simulink model "Energy_Management_Model1"  (R2025a)
settings: Solver=ode4  StartTime=0.0  StopTime=86400  FixedStep=3600  RelTol=1e-3
values from neighbouring files (symbols this model uses):
  A = 150    [setup_parameters.m]
  C_bat = 10    [setup_parameters.m]
  eta = 0.18    [setup_parameters.m]
  P_bat_max = 2    [setup_parameters.m]
  SOC_init = [0.3, 0.6, 0.9]    [setup_parameters.m]
  SOC_max = 0.98    [setup_parameters.m]
  SOC_min = 0.2    [setup_parameters.m]
  Ts = 3600    [setup_parameters.m]
libraries: simulink x3
settings Model: Creator=ENG HOSAM  LastModifiedBy=mtabrez
settings SolverCC: AlgebraicLoopSolver=TrustRegion
settings DebuggingCC: UnconnectedInputMsg=warning  UnconnectedOutputMsg=warning  UnconnectedLineMsg=warning
settings ModelReferenceCC: EnableRefExpFcnMdlSchedulingChecks=on
settings RTWCC: GPUComputeCapability=3.5

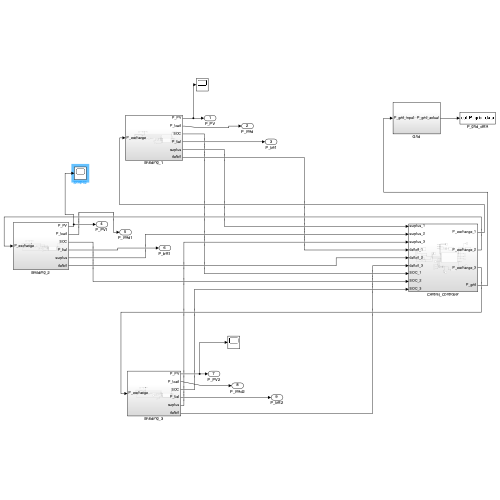
[thumbnail: Simulink's stored preview of the top-level diagram]
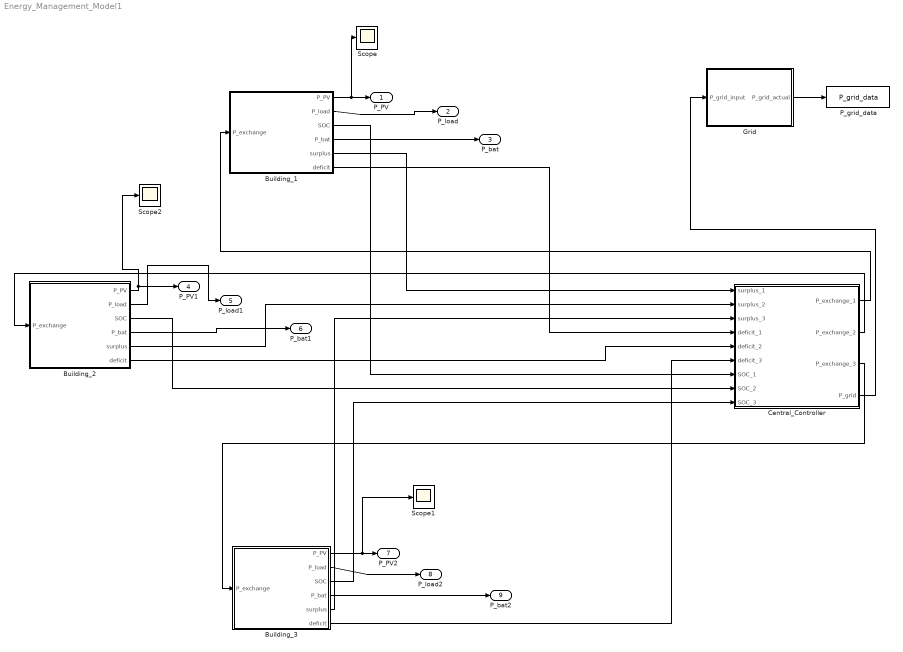
== system Energy_Management_Model1 ==
  Building_1 : Subsystem
  Building_2 : Subsystem
  Building_3 : Subsystem
  Central_Controller : Subsystem
  Grid : Subsystem
  P_grid_data : ToWorkspace  VariableName=P_grid_data  SampleTime=-1
  Scope : Scope
      settings: ActiveDisplayYMinimum=-3.3749999999999991  ActiveDisplayYMaximum=30.375  DataLoggingVariableName=ScopeData5
  Scope1 : Scope
      settings: DataLoggingVariableName=ScopeData6
  Scope2 : Scope
      settings: ActiveDisplayYMinimum=-3.3749999999999991  ActiveDisplayYMaximum=30.375  DataLoggingVariableName=ScopeData7
  P_PV : Outport
  P_load : Outport  Port=2
  P_bat : Outport  Port=3
  P_PV1 : Outport  Port=4
  P_load1 : Outport  Port=5
  P_bat1 : Outport  Port=6
  P_PV2 : Outport  Port=7
  P_load2 : Outport  Port=8
  P_bat2 : Outport  Port=9
  wires:
  Building_1/1(P_PV) -> Scope/1, P_PV/1
  Building_1/2(P_load) -> P_load/1
  Building_1/4(P_bat) -> P_bat/1
  Building_2/4(P_bat) -> P_bat1/1
  Building_2/1(P_PV) -> P_PV1/1, Scope2/1
  Building_2/2(P_load) -> P_load1/1
  Building_3/4(P_bat) -> P_bat2/1
  Building_3/1(P_PV) -> Scope1/1, P_PV2/1
  Building_3/2(P_load) -> P_load2/1
  Building_1/5(surplus) -> Central_Controller/1(surplus_1)
  Building_2/5(surplus) -> Central_Controller/2(surplus_2)
  Building_3/5(surplus) -> Central_Controller/3(surplus_3)
  Building_1/6(deficit) -> Central_Controller/4(deficit_1)
  Building_2/6(deficit) -> Central_Controller/5(deficit_2)
  Building_3/6(deficit) -> Central_Controller/6(deficit_3)
  Building_1/3(SOC) -> Central_Controller/7(SOC_1)
  Building_2/3(SOC) -> Central_Controller/8(SOC_2)
  Building_3/3(SOC) -> Central_Controller/9(SOC_3)
  Central_Controller/1(P_exchange_1) -> Building_1/1(P_exchange)
  Central_Controller/2(P_exchange_2) -> Building_2/1(P_exchange)
  Central_Controller/3(P_exchange_3) -> Building_3/1(P_exchange)
  Central_Controller/4(P_grid) -> Grid/1(P_grid_input)
  Grid/1(P_grid_actual) -> P_grid_data/1

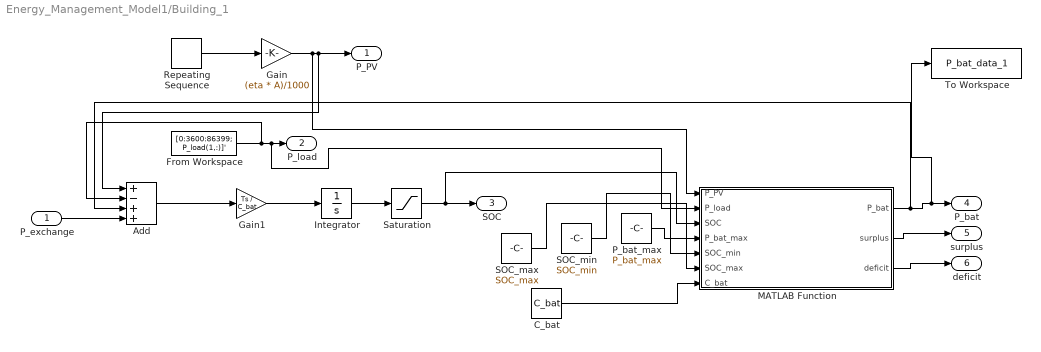
== system Energy_Management_Model1/Building_1 ==
  P_exchange : Inport
  Add : Sum  Inputs=+-++
  C_bat : Constant  Value=C_bat
  From Workspace : FromWorkspace  VariableName=[0:3600:86399; P_load(1,:)]'  OutDataTypeStr=double
  Gain : Gain  Gain=(eta * A)/1000
  Gain1 : Gain  Gain=Ts / C_bat
  Integrator : Integrator  InitialCondition=SOC_init(1)
  MATLAB Function : MATLAB Function  TreatAsAtomicUnit=on
  P_bat_max : Constant  Value=P_bat_max
  Repeating Sequence : simulink/Sources/Repeating Sequence  rep_seq_t=0:3600:82800  rep_seq_y=G
  SOC_max : Constant  Value=SOC_max
  SOC_min : Constant  Value=SOC_min
  Saturation : Saturate  UpperLimit=SOC_max  LowerLimit=SOC_min
  To Workspace : ToWorkspace  VariableName=P_bat_data_1  SampleTime=-1
  P_PV : Outport
  P_load : Outport  Port=2
  SOC : Outport  Port=3
  P_bat : Outport  Port=4
  surplus : Outport  Port=5
  deficit : Outport  Port=6
  wires:
  Integrator/1 -> Saturation/1
  MATLAB Function/3(deficit) -> deficit/1
  Gain1/1 -> Integrator/1
  From Workspace/1 -> Add/2, P_load/1, MATLAB Function/2(P_load)
  Gain/1 -> Add/1, P_PV/1, MATLAB Function/1(P_PV)
  Repeating Sequence/1 -> Gain/1
  Saturation/1 -> SOC/1, MATLAB Function/3(SOC)
  P_bat_max/1 -> MATLAB Function/4(P_bat_max)
  MATLAB Function/1(P_bat) -> Add/3, To Workspace/1, P_bat/1
  MATLAB Function/2(surplus) -> surplus/1
  SOC_max/1 -> MATLAB Function/6(SOC_max)
  SOC_min/1 -> MATLAB Function/5(SOC_min)
  C_bat/1 -> MATLAB Function/7(C_bat)
  Add/1 -> Gain1/1
  P_exchange/1 -> Add/4

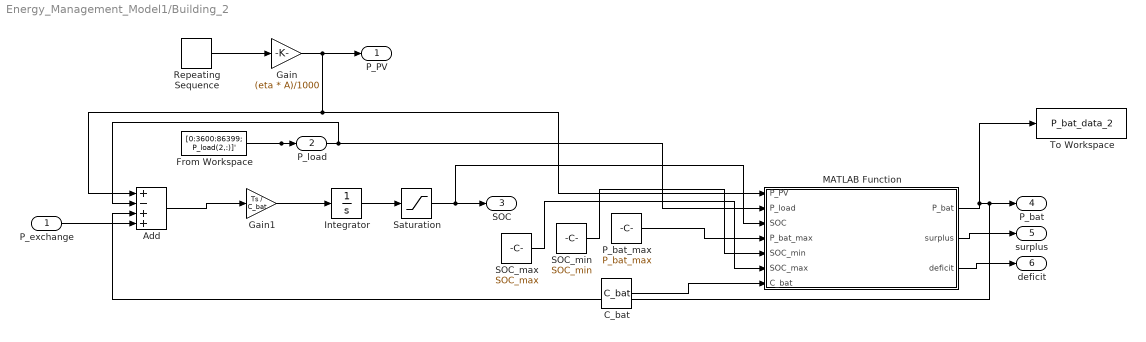
== system Energy_Management_Model1/Building_2 ==
  P_exchange : Inport
  Add : Sum  Inputs=+-++
  C_bat : Constant  Value=C_bat
  From Workspace : FromWorkspace  VariableName=[0:3600:86399; P_load(2,:)]'  OutDataTypeStr=double
  Gain : Gain  Gain=(eta * A)/1000
  Gain1 : Gain  Gain=Ts / C_bat
  Integrator : Integrator  InitialCondition=SOC_init(2)
  MATLAB Function : MATLAB Function  TreatAsAtomicUnit=on
  P_bat_max : Constant  Value=P_bat_max
  Repeating Sequence : simulink/Sources/Repeating Sequence  rep_seq_t=0:3600:82800  rep_seq_y=G
  SOC_max : Constant  Value=SOC_max
  SOC_min : Constant  Value=SOC_min
  Saturation : Saturate  UpperLimit=SOC_max  LowerLimit=SOC_min
  To Workspace : ToWorkspace  VariableName=P_bat_data_2  SampleTime=-1
  P_PV : Outport
  P_load : Outport  Port=2
  SOC : Outport  Port=3
  P_bat : Outport  Port=4
  surplus : Outport  Port=5
  deficit : Outport  Port=6
  wires:
  Integrator/1 -> Saturation/1
  MATLAB Function/3(deficit) -> deficit/1
  MATLAB Function/1(P_bat) -> To Workspace/1, Add/3, P_bat/1
  Gain1/1 -> Integrator/1
  From Workspace/1 -> P_load/1, Add/2, MATLAB Function/2(P_load)
  Gain/1 -> P_PV/1, Add/1, MATLAB Function/1(P_PV)
  Repeating Sequence/1 -> Gain/1
  Saturation/1 -> SOC/1, MATLAB Function/3(SOC)
  P_bat_max/1 -> MATLAB Function/4(P_bat_max)
  Add/1 -> Gain1/1
  MATLAB Function/2(surplus) -> surplus/1
  SOC_max/1 -> MATLAB Function/6(SOC_max)
  SOC_min/1 -> MATLAB Function/5(SOC_min)
  P_exchange/1 -> Add/4
  C_bat/1 -> MATLAB Function/7(C_bat)

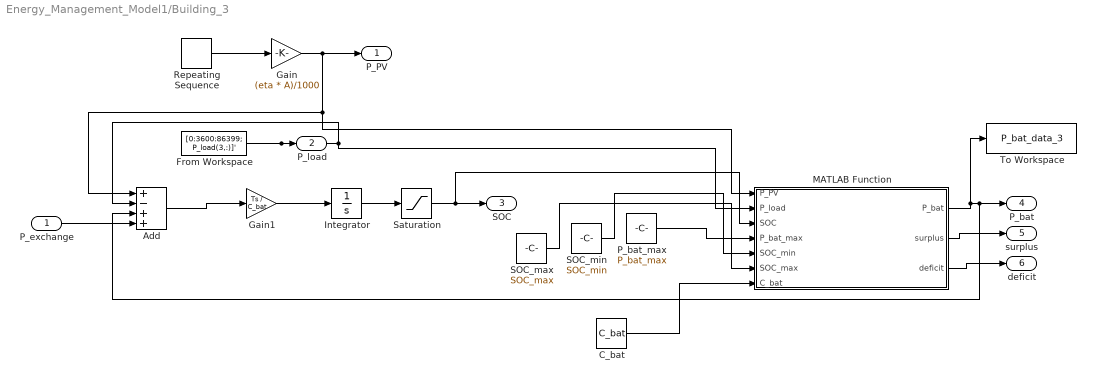
== system Energy_Management_Model1/Building_3 ==
  P_exchange : Inport
  Add : Sum  Inputs=+-++
  C_bat : Constant  Value=C_bat
  From Workspace : FromWorkspace  VariableName=[0:3600:86399; P_load(3,:)]'  OutDataTypeStr=double
  Gain : Gain  Gain=(eta * A)/1000
  Gain1 : Gain  Gain=Ts / C_bat
  Integrator : Integrator  InitialCondition=SOC_init(3)
  MATLAB Function : MATLAB Function  TreatAsAtomicUnit=on
  P_bat_max : Constant  Value=P_bat_max
  Repeating Sequence : simulink/Sources/Repeating Sequence  rep_seq_t=0:3600:82800  rep_seq_y=G
  SOC_max : Constant  Value=SOC_max
  SOC_min : Constant  Value=SOC_min
  Saturation : Saturate  UpperLimit=SOC_max  LowerLimit=SOC_min
  To Workspace : ToWorkspace  VariableName=P_bat_data_3  SampleTime=-1
  P_PV : Outport
  P_load : Outport  Port=2
  SOC : Outport  Port=3
  P_bat : Outport  Port=4
  surplus : Outport  Port=5
  deficit : Outport  Port=6
  wires:
  Integrator/1 -> Saturation/1
  MATLAB Function/3(deficit) -> deficit/1
  MATLAB Function/1(P_bat) -> To Workspace/1, Add/3, P_bat/1
  Gain1/1 -> Integrator/1
  From Workspace/1 -> P_load/1, Add/2, MATLAB Function/2(P_load)
  Gain/1 -> P_PV/1, Add/1, MATLAB Function/1(P_PV)
  Repeating Sequence/1 -> Gain/1
  Saturation/1 -> SOC/1, MATLAB Function/3(SOC)
  P_bat_max/1 -> MATLAB Function/4(P_bat_max)
  Add/1 -> Gain1/1
  MATLAB Function/2(surplus) -> surplus/1
  SOC_max/1 -> MATLAB Function/6(SOC_max)
  SOC_min/1 -> MATLAB Function/5(SOC_min)
  P_exchange/1 -> Add/4
  C_bat/1 -> MATLAB Function/7(C_bat)

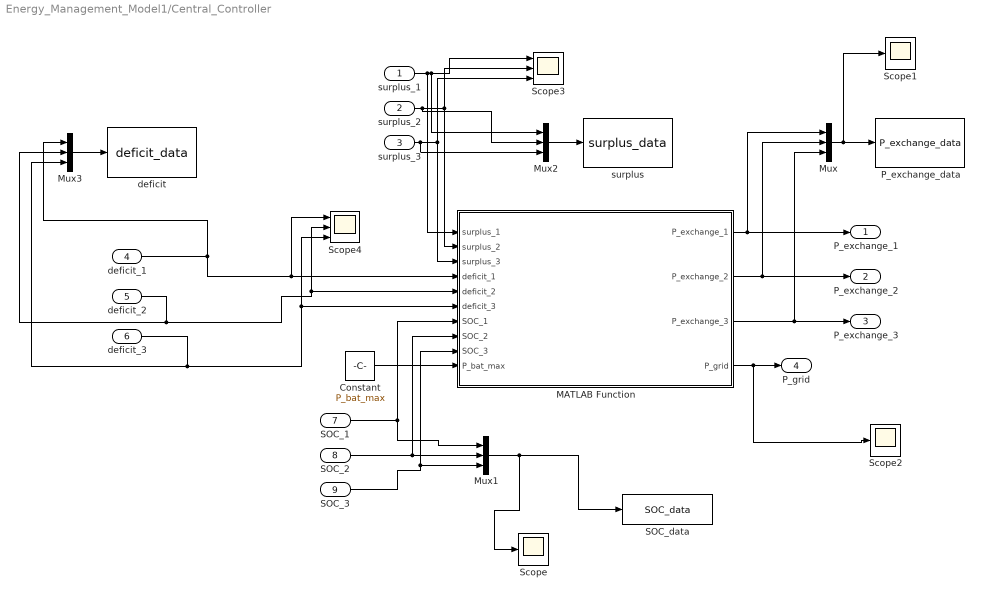
== system Energy_Management_Model1/Central_Controller ==
  surplus_1 : Inport
  surplus_2 : Inport  Port=2
  surplus_3 : Inport  Port=3
  deficit_1 : Inport  Port=4
  deficit_2 : Inport  Port=5
  deficit_3 : Inport  Port=6
  SOC_1 : Inport  Port=7
  SOC_2 : Inport  Port=8
  SOC_3 : Inport  Port=9
  Constant : Constant  Value=P_bat_max
  MATLAB Function : MATLAB Function  TreatAsAtomicUnit=on
  Mux{,1..3} (4 alike) : Mux  Inputs=3
  P_exchange_data : ToWorkspace  VariableName=P_exchange_data  SampleTime=-1
  SOC_data : ToWorkspace  VariableName=SOC_data  SampleTime=-1
  Scope : Scope
      settings: ActiveDisplayYMinimum=0.1025  ActiveDisplayYMaximum=1.0775
  Scope1 : Scope
      settings: ActiveDisplayYMinimum=-0.25  ActiveDisplayYMaximum=2.25
  Scope2 : Scope
      settings: ActiveDisplayYMinimum=-16.425  ActiveDisplayYMaximum=87.825  DataLoggingVariableName=ScopeData2
  Scope3 : Scope  NumInputPorts=3
      settings: ActiveDisplayYMinimum=-3.2375  ActiveDisplayYMaximum=29.1375  DataLoggingVariableName=ScopeData3
  Scope4 : Scope  NumInputPorts=3
      settings: ActiveDisplayYMinimum=-0.275  ActiveDisplayYMaximum=2.475  DataLoggingVariableName=ScopeData4
  deficit : ToWorkspace  VariableName=deficit_data  SampleTime=-1
  surplus : ToWorkspace  VariableName=surplus_data  SampleTime=-1
  P_exchange_1 : Outport
  P_exchange_2 : Outport  Port=2
  P_exchange_3 : Outport  Port=3
  P_grid : Outport  Port=4
  wires:
  SOC_2/1 -> MATLAB Function/8(SOC_2), Mux1/2
  SOC_1/1 -> MATLAB Function/7(SOC_1), Mux1/1
  MATLAB Function/1(P_exchange_1) -> Mux/1, P_exchange_1/1
  SOC_3/1 -> MATLAB Function/9(SOC_3), Mux1/3
  Mux1/1 -> Scope/1, SOC_data/1
  MATLAB Function/3(P_exchange_3) -> Mux/3, P_exchange_3/1
  MATLAB Function/2(P_exchange_2) -> Mux/2, P_exchange_2/1
  Mux/1 -> Scope1/1, P_exchange_data/1
  surplus_2/1 -> Mux2/2, Scope3/2, MATLAB Function/2(surplus_2)
  surplus_3/1 -> Mux2/3, Scope3/3, MATLAB Function/3(surplus_3)
  deficit_1/1 -> Mux3/1, Scope4/1, MATLAB Function/4(deficit_1)
  deficit_2/1 -> Scope4/2, MATLAB Function/5(deficit_2), Mux3/2
  deficit_3/1 -> MATLAB Function/6(deficit_3), Scope4/3, Mux3/3
  MATLAB Function/4(P_grid) -> Scope2/1, P_grid/1
  surplus_1/1 -> Mux2/1, Scope3/1, MATLAB Function/1(surplus_1)
  Mux2/1 -> surplus/1
  Mux3/1 -> deficit/1
  Constant/1 -> MATLAB Function/10(P_bat_max)

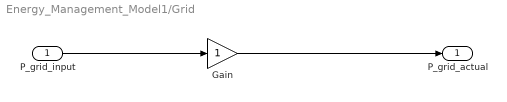
== system Energy_Management_Model1/Grid ==
  P_grid_input : Inport
  Gain : Gain
  P_grid_actual : Outport
  wires:
  P_grid_input/1 -> Gain/1
  Gain/1 -> P_grid_actual/1

== matlab function Energy_Management_Model1/Building_2/MATLAB Function ==
  data: P_PV input; P_bat output; P_load input; SOC input; P_bat_max input; SOC_min input; SOC_max input; surplus output; deficit output; C_bat input
function [P_bat, surplus, deficit] = local_controller(P_PV, P_load, SOC, P_bat_max, SOC_min, SOC_max, C_bat)
    net_power = P_PV - P_load;
    P_bat = 0;
    surplus = 0;
    deficit = 0;
    
    if net_power > 0
        if SOC < 0.8 && SOC < 0.98
            max_charge = min(P_bat_max, (SOC_max - SOC) * C_bat);
            P_bat = min(net_power, max_charge);
        end
        surplus = max(0, net_power - P_bat);
    elseif net_power < 0
        if SOC > 0.3 || (SOC > 0.7 && net_power < -0.1)
            max_discharge = min(P_bat_max, (SOC - SOC_min) * C_bat);
            P_bat = max(net_power, -max_discharge);
        end
        deficit = max(0, -net_power - P_bat);
    end
end

== matlab function Energy_Management_Model1/Building_1/MATLAB Function ==
  data: P_PV input; P_bat output; P_load input; SOC input; P_bat_max input; SOC_min input; SOC_max input; surplus output; deficit output; C_bat input
function [P_bat, surplus, deficit] = local_controller(P_PV, P_load, SOC, P_bat_max, SOC_min, SOC_max, C_bat)
    net_power = P_PV - P_load;
    P_bat = 0;
    surplus = 0;
    deficit = 0;
    
    if net_power > 0
        if SOC < 0.8 && SOC < 0.98
            max_charge = min(P_bat_max, (SOC_max - SOC) * C_bat);
            P_bat = min(net_power, max_charge);
        end
        surplus = max(0, net_power - P_bat);
    elseif net_power < 0
        if SOC > 0.3 || (SOC > 0.7 && net_power < -0.1)
            max_discharge = min(P_bat_max, (SOC - SOC_min) * C_bat);
            P_bat = max(net_power, -max_discharge);
        end
        deficit = max(0, -net_power - P_bat);
    end
end

== matlab function Energy_Management_Model1/Building_3/MATLAB Function ==
  data: P_PV input; P_bat output; P_load input; SOC input; P_bat_max input; SOC_min input; SOC_max input; surplus output; deficit output; C_bat input
function [P_bat, surplus, deficit] = local_controller(P_PV, P_load, SOC, P_bat_max, SOC_min, SOC_max, C_bat)
    net_power = P_PV - P_load;
    P_bat = 0;
    surplus = 0;
    deficit = 0;
    
    if net_power > 0
        if SOC < 0.8 && SOC < 0.98
            max_charge = min(P_bat_max, (SOC_max - SOC) * C_bat);
            P_bat = min(net_power, max_charge);
        end
        surplus = max(0, net_power - P_bat);
    elseif net_power < 0
        if SOC > 0.3 || (SOC > 0.7 && net_power < -0.1)
            max_discharge = min(P_bat_max, (SOC - SOC_min) * C_bat);
            P_bat = max(net_power, -max_discharge);
        end
        deficit = max(0, -net_power - P_bat);
    end
end

== matlab function Energy_Management_Model1/Central_Controller/MATLAB Function ==
  data: surplus_1 input; P_exchange_1 output; P_exchange_2 output; P_exchange_3 output; surplus_2 input; surplus_3 input; deficit_1 input; deficit_2 input; deficit_3 input; SOC_1 input; SOC_2 input; SOC_3 input; P_grid output; P_bat_max input
function [P_exchange_1, P_exchange_2, P_exchange_3, P_grid] = central_controller(...
    surplus_1, surplus_2, surplus_3, ...
    deficit_1, deficit_2, deficit_3, ...
    SOC_1, SOC_2, SOC_3, P_bat_max)
    
    surplus = [surplus_1; surplus_2; surplus_3];
    deficit = [deficit_1; deficit_2; deficit_3];
    SOC = [SOC_1; SOC_2; SOC_3];
    
    P_exchange = zeros(3, 1);
    
    total_surplus = sum(surplus);
    total_deficit = sum(deficit);
    
    if total_surplus > 0.1 && total_deficit > 0.1
        available_energy = min(total_surplus, total_deficit);
        
        for i = 1:3
            if surplus(i) > 0.01 && SOC(i) < 0.9
                contribution_ratio = surplus(i) / total_surplus;
                P_exchange(i) = -min(available_energy * contribution_ratio, P_bat_max);
            end
        end
        
        for j = 1:3
            if deficit(j) > 0.01 && SOC(j) > 0.3
                need_ratio = deficit(j) / total_deficit;
                P_exchange(j) = min(available_energy * need_ratio, P_bat_max);
            end
        end
    end
    
    if total_surplus > 0.1 && total_deficit <= 0.1
        for i = 1:3
            if surplus(i) > 0.01 && SOC(i) < 0.9
                P_exchange(i) = -min(surplus(i), P_bat_max);
            end
        end
    end
    
    if total_surplus <= 0.1 && total_deficit > 0.1
        for j = 1:3
            if deficit(j) > 0.01 && SOC(j) > 0.3
                P_exchange(j) = min(deficit(j), P_bat_max);
            end
        end
    end
    
    P_grid = total_surplus - total_deficit;
    
    P_exchange_1 = P_exchange(1);
    P_exchange_2 = P_exchange(2);
    P_exchange_3 = P_exchange(3);
end
